simulink model "My_gfm_battery_sil_2"  (R2018b)
settings: Solver=ode45  StartTime=0.0  StopTime=30  MaxStep=1e-4  RelTol=1e-3
PreLoadFcn:
  | modelDir = fileparts(get_param(bdroot,'FileName'));
  | 
  | load_system(fullfile(modelDir,'controls_element_lib.slx'));
  | load_system(fullfile(modelDir,'test_sequence_lib.slx'));
InitFcn:
  | close all;
  | clear all;
  | clc;
  | 
  | % frequency nominals
  | F_NOM = 60;
  | W_NOM = 2 * pi * F_NOM;
  | 
  | % base values relative to inverter
  | % --------------------------------
  | VLL_INV_NOM = 480;
  | P_INV_NOM = 1e6;
  | Q_INV_NOM = 0.5e6;
  | S_INV_NOM = sqrt(P_INV_NOM^2 + Q_INV_NOM^2);
  | 
  | I_INV_BASE = S_INV_NOM/(sqrt(3)*VLL_INV_NOM);
  | Z_INV_BASE = VLL_INV_NOM^2/S_INV_NOM;
  | L_INV_BASE = Z_INV_BASE / W_NOM;
  | C_INV_BASE = 1 / (Z_INV_BASE * W_NOM);
  | 
  | % nominal ratings for Plant model
  | % --------------------------------------
  | INVERTER_COUNT = 100;
  | 
  | VLV_NOM = VLL_INV_NOM;
  | VMV_NOM = 35e3;
  | VHV_NOM = 230e3;
  | S_PLANT = INVERTER_COUNT * S_INV_NOM;
  | 
  | N_GSU = VHV_NOM/VMV_NOM;
  | N_MVT = VMV_NOM/VLV_NOM;
  | 
  | I_LV_BASE = S_PLANT/(sqrt(3)*VLV_NOM);
  | I_MV_BASE = S_PLANT/(sqrt(3)*VMV_NOM);
  | I_HV_BASE = S_PLANT/(sqrt(3)*VHV_NOM);
  | 
  | Z_LV_BASE = VLV_NOM^2/S_PLANT;
  | Z_MV_BASE = VMV_NOM^2/S_PLANT;
  | Z_HV_BASE = VHV_NOM^2/S_PLANT;
  | 
  | L_LV_BASE = Z_LV_BASE / W_NOM;
  | L_MV_BASE = Z_MV_BASE / W_NOM;
  | L_HV_BASE = Z_HV_BASE / W_NOM;
  | C_LV_BASE = 1 / (Z_LV_BASE * W_NOM);
  | C_MV_BASE = 1 / (Z_MV_BASE * W_NOM);
  | C_HV_BASE = 1 / (Z_HV_BASE * W_NOM);
  | 
  | % nominal ratings for Grid model
  | % --------------------------------------
  | VGRID_NOM = VHV_NOM;
  | S_GRID = 2*S_PLANT;
  | I_HV_BASE = S_GRID/(sqrt(3)*VGRID_NOM);
  | Z_GRID_BASE = VGRID_NOM^2/S_GRID;
  | L_GRID_BASE = Z_GRID_BASE / W_NOM;
  | C_GRID_BASE = 1 / (Z_GRID_BASE * W_NOM);
undefined symbols (not defined in the file): j
libraries: simulink x74, controls_element_lib x20, test_sequence_lib x12
(part 5 of 9)

== system My_gfm_battery_sil_2/My Inverter Controller /My_acChecks_A_V3/Clear Timer5 ==
  note: Max one sample delay on Rise
  note: Min one sample delay on Fall
  in : Inport
  Constant : Constant  Value=T_STEP
  Constant1 : Constant  Value=0
  Constant2 : Constant  Value=TIMEOUT
  Constant3 : Constant  Value=T_STEP
  Min1 : MinMax  Function=max  Inputs=2
  Min2 : MinMax  Function=max  Inputs=2
  Relational Operator : RelationalOperator  Operator=>  OutDataTypeStr=boolean  RndMeth=Simplest
  Sum1 : Sum  Inputs=|++
  Sum2 : Sum  Inputs=|-+
  Switch : Switch  Criteria=u2 > Threshold
  Unit Delay : UnitDelay  InitialCondition=TIMER_INIT  SampleTime=T_STEP
  out : Outport  VectorParamsAs1DForOutWhenUnconnected=on
  wires:
  Sum1/1 -> Switch/1
  Sum2/1 -> Relational Operator/1, Min2/1
  Constant/1 -> Sum2/1
  Min2/1 -> Switch/3
  Constant1/1 -> Min2/2, Relational Operator/2
  Unit Delay/1 -> Sum2/2
  in/1 -> Switch/2
  Switch/1 -> Unit Delay/1
  Relational Operator/1 -> out/1
  Constant2/1 -> Min1/1
  Constant3/1 -> Min1/2, Sum1/2
  Min1/1 -> Sum1/1

== system My_gfm_battery_sil_2/My Inverter Controller /My_acChecks_A_V3/Clear Timer6 ==
  note: Max one sample delay on Rise
  note: Min one sample delay on Fall
  in : Inport
  Constant : Constant  Value=T_STEP
  Constant1 : Constant  Value=0
  Constant2 : Constant  Value=TIMEOUT
  Constant3 : Constant  Value=T_STEP
  Min1 : MinMax  Function=max  Inputs=2
  Min2 : MinMax  Function=max  Inputs=2
  Relational Operator : RelationalOperator  Operator=>  OutDataTypeStr=boolean  RndMeth=Simplest
  Sum1 : Sum  Inputs=|++
  Sum2 : Sum  Inputs=|-+
  Switch : Switch  Criteria=u2 > Threshold
  Unit Delay : UnitDelay  InitialCondition=TIMER_INIT  SampleTime=T_STEP
  out : Outport  VectorParamsAs1DForOutWhenUnconnected=on
  wires:
  Sum1/1 -> Switch/1
  Sum2/1 -> Relational Operator/1, Min2/1
  Constant/1 -> Sum2/1
  Min2/1 -> Switch/3
  Constant1/1 -> Min2/2, Relational Operator/2
  Unit Delay/1 -> Sum2/2
  in/1 -> Switch/2
  Switch/1 -> Unit Delay/1
  Relational Operator/1 -> out/1
  Constant2/1 -> Min1/1
  Constant3/1 -> Min1/2, Sum1/2
  Min1/1 -> Sum1/1

== system My_gfm_battery_sil_2/My Inverter Controller /My_acChecks_A_V3/Clear Timer7 ==
  note: Max one sample delay on Rise
  note: Min one sample delay on Fall
  in : Inport
  Constant : Constant  Value=T_STEP
  Constant1 : Constant  Value=0
  Constant2 : Constant  Value=TIMEOUT
  Constant3 : Constant  Value=T_STEP
  Min1 : MinMax  Function=max  Inputs=2
  Min2 : MinMax  Function=max  Inputs=2
  Relational Operator : RelationalOperator  Operator=>  OutDataTypeStr=boolean  RndMeth=Simplest
  Sum1 : Sum  Inputs=|++
  Sum2 : Sum  Inputs=|-+
  Switch : Switch  Criteria=u2 > Threshold
  Unit Delay : UnitDelay  InitialCondition=TIMER_INIT  SampleTime=T_STEP
  out : Outport  VectorParamsAs1DForOutWhenUnconnected=on
  wires:
  Sum1/1 -> Switch/1
  Sum2/1 -> Relational Operator/1, Min2/1
  Constant/1 -> Sum2/1
  Min2/1 -> Switch/3
  Constant1/1 -> Min2/2, Relational Operator/2
  Unit Delay/1 -> Sum2/2
  in/1 -> Switch/2
  Switch/1 -> Unit Delay/1
  Relational Operator/1 -> out/1
  Constant2/1 -> Min1/1
  Constant3/1 -> Min1/2, Sum1/2
  Min1/1 -> Sum1/1

== system My_gfm_battery_sil_2/My Inverter Controller /My_acChecks_A_V3/Clear Timer8 ==
  note: Max one sample delay on Rise
  note: Min one sample delay on Fall
  in : Inport
  Constant : Constant  Value=T_STEP
  Constant1 : Constant  Value=0
  Constant2 : Constant  Value=TIMEOUT
  Constant3 : Constant  Value=T_STEP
  Min1 : MinMax  Function=max  Inputs=2
  Min2 : MinMax  Function=max  Inputs=2
  Relational Operator : RelationalOperator  Operator=>  OutDataTypeStr=boolean  RndMeth=Simplest
  Sum1 : Sum  Inputs=|++
  Sum2 : Sum  Inputs=|-+
  Switch : Switch  Criteria=u2 > Threshold
  Unit Delay : UnitDelay  InitialCondition=TIMER_INIT  SampleTime=T_STEP
  out : Outport  VectorParamsAs1DForOutWhenUnconnected=on
  wires:
  Sum1/1 -> Switch/1
  Sum2/1 -> Relational Operator/1, Min2/1
  Constant/1 -> Sum2/1
  Min2/1 -> Switch/3
  Constant1/1 -> Min2/2, Relational Operator/2
  Unit Delay/1 -> Sum2/2
  in/1 -> Switch/2
  Switch/1 -> Unit Delay/1
  Relational Operator/1 -> out/1
  Constant2/1 -> Min1/1
  Constant3/1 -> Min1/2, Sum1/2
  Min1/1 -> Sum1/1

== system My_gfm_battery_sil_2/My Inverter Controller /My_acChecks_A_V3/Clear Timer9 ==
  note: Max one sample delay on Rise
  note: Min one sample delay on Fall
  in : Inport
  Constant : Constant  Value=T_STEP
  Constant1 : Constant  Value=0
  Constant2 : Constant  Value=TIMEOUT
  Constant3 : Constant  Value=T_STEP
  Min1 : MinMax  Function=max  Inputs=2
  Min2 : MinMax  Function=max  Inputs=2
  Relational Operator : RelationalOperator  Operator=>  OutDataTypeStr=boolean  RndMeth=Simplest
  Sum1 : Sum  Inputs=|++
  Sum2 : Sum  Inputs=|-+
  Switch : Switch  Criteria=u2 > Threshold
  Unit Delay : UnitDelay  InitialCondition=TIMER_INIT  SampleTime=T_STEP
  out : Outport  VectorParamsAs1DForOutWhenUnconnected=on
  wires:
  Sum1/1 -> Switch/1
  Sum2/1 -> Relational Operator/1, Min2/1
  Constant/1 -> Sum2/1
  Min2/1 -> Switch/3
  Constant1/1 -> Min2/2, Relational Operator/2
  Unit Delay/1 -> Sum2/2
  in/1 -> Switch/2
  Switch/1 -> Unit Delay/1
  Relational Operator/1 -> out/1
  Constant2/1 -> Min1/1
  Constant3/1 -> Min1/2, Sum1/2
  Min1/1 -> Sum1/1

== system My_gfm_battery_sil_2/My Inverter Controller /My_acChecks_A_V3/OF1 Timer ==
  note: Min one sample delay on Rise
  note: Max one sample delay on Fall
  in : Inport
  Constant : Constant  Value=T_STEP
  Constant1 : Constant  Value=0
  Constant2 : Constant  Value=TIMEOUT
  Constant3 : Constant  Value=T_STEP
  Gain : Gain  Gain=0
  Min1 : MinMax  Function=max  Inputs=2
  Min2 : MinMax  Inputs=2
  Relational Operator : RelationalOperator  Operator=>  OutDataTypeStr=boolean  RndMeth=Simplest
  Sum1 : Sum  Inputs=|++
  Sum2 : Sum  Inputs=|++
  Switch : Switch  Criteria=u2 > Threshold
  Unit Delay : UnitDelay  SampleTime=T_STEP
  out : Outport  VectorParamsAs1DForOutWhenUnconnected=on
  wires:
  Sum2/1 -> Relational Operator/1, Min2/1
  Sum1/1 -> Min2/2, Relational Operator/2
  Constant/1 -> Sum2/1
  Min2/1 -> Switch/1
  Constant1/1 -> Switch/3
  Unit Delay/1 -> Sum2/2
  in/1 -> Switch/2
  Switch/1 -> Unit Delay/1
  Relational Operator/1 -> out/1
  Min1/1 -> Sum1/1
  Constant2/1 -> Min1/1
  Constant3/1 -> Min1/2, Gain/1
  Gain/1 -> Sum1/2

== system My_gfm_battery_sil_2/My Inverter Controller /My_acChecks_A_V3/OF2 Timer ==
  note: Min one sample delay on Rise
  note: Max one sample delay on Fall
  in : Inport
  Constant : Constant  Value=T_STEP
  Constant1 : Constant  Value=0
  Constant2 : Constant  Value=TIMEOUT
  Constant3 : Constant  Value=T_STEP
  Gain : Gain  Gain=0
  Min1 : MinMax  Function=max  Inputs=2
  Min2 : MinMax  Inputs=2
  Relational Operator : RelationalOperator  Operator=>  OutDataTypeStr=boolean  RndMeth=Simplest
  Sum1 : Sum  Inputs=|++
  Sum2 : Sum  Inputs=|++
  Switch : Switch  Criteria=u2 > Threshold
  Unit Delay : UnitDelay  SampleTime=T_STEP
  out : Outport  VectorParamsAs1DForOutWhenUnconnected=on
  wires:
  Sum2/1 -> Relational Operator/1, Min2/1
  Sum1/1 -> Min2/2, Relational Operator/2
  Constant/1 -> Sum2/1
  Min2/1 -> Switch/1
  Constant1/1 -> Switch/3
  Unit Delay/1 -> Sum2/2
  in/1 -> Switch/2
  Switch/1 -> Unit Delay/1
  Relational Operator/1 -> out/1
  Min1/1 -> Sum1/1
  Constant2/1 -> Min1/1
  Constant3/1 -> Min1/2, Gain/1
  Gain/1 -> Sum1/2

== system My_gfm_battery_sil_2/My Inverter Controller /My_acChecks_A_V3/OF3 Timer ==
  note: Min one sample delay on Rise
  note: Max one sample delay on Fall
  in : Inport
  Constant : Constant  Value=T_STEP
  Constant1 : Constant  Value=0
  Constant2 : Constant  Value=TIMEOUT
  Constant3 : Constant  Value=T_STEP
  Gain : Gain  Gain=0
  Min1 : MinMax  Function=max  Inputs=2
  Min2 : MinMax  Inputs=2
  Relational Operator : RelationalOperator  Operator=>  OutDataTypeStr=boolean  RndMeth=Simplest
  Sum1 : Sum  Inputs=|++
  Sum2 : Sum  Inputs=|++
  Switch : Switch  Criteria=u2 > Threshold
  Unit Delay : UnitDelay  SampleTime=T_STEP
  out : Outport  VectorParamsAs1DForOutWhenUnconnected=on
  wires:
  Sum2/1 -> Relational Operator/1, Min2/1
  Sum1/1 -> Min2/2, Relational Operator/2
  Constant/1 -> Sum2/1
  Min2/1 -> Switch/1
  Constant1/1 -> Switch/3
  Unit Delay/1 -> Sum2/2
  in/1 -> Switch/2
  Switch/1 -> Unit Delay/1
  Relational Operator/1 -> out/1
  Min1/1 -> Sum1/1
  Constant2/1 -> Min1/1
  Constant3/1 -> Min1/2, Gain/1
  Gain/1 -> Sum1/2

== system My_gfm_battery_sil_2/My Inverter Controller /My_acChecks_A_V3/OV1 Timer ==
  note: Min one sample delay on Rise
  note: Max one sample delay on Fall
  in : Inport
  Constant : Constant  Value=T_STEP
  Constant1 : Constant  Value=0
  Constant2 : Constant  Value=TIMEOUT
  Constant3 : Constant  Value=T_STEP
  Gain : Gain  Gain=0
  Min1 : MinMax  Function=max  Inputs=2
  Min2 : MinMax  Inputs=2
  Relational Operator : RelationalOperator  Operator=>  OutDataTypeStr=boolean  RndMeth=Simplest
  Sum1 : Sum  Inputs=|++
  Sum2 : Sum  Inputs=|++
  Switch : Switch  Criteria=u2 > Threshold
  Unit Delay : UnitDelay  SampleTime=T_STEP
  out : Outport  VectorParamsAs1DForOutWhenUnconnected=on
  wires:
  Sum2/1 -> Relational Operator/1, Min2/1
  Sum1/1 -> Min2/2, Relational Operator/2
  Constant/1 -> Sum2/1
  Min2/1 -> Switch/1
  Constant1/1 -> Switch/3
  Unit Delay/1 -> Sum2/2
  in/1 -> Switch/2
  Switch/1 -> Unit Delay/1
  Relational Operator/1 -> out/1
  Min1/1 -> Sum1/1
  Constant2/1 -> Min1/1
  Constant3/1 -> Min1/2, Gain/1
  Gain/1 -> Sum1/2

== system My_gfm_battery_sil_2/My Inverter Controller /My_acChecks_A_V3/OV2 Timer ==
  note: Min one sample delay on Rise
  note: Max one sample delay on Fall
  in : Inport
  Constant : Constant  Value=T_STEP
  Constant1 : Constant  Value=0
  Constant2 : Constant  Value=TIMEOUT
  Constant3 : Constant  Value=T_STEP
  Gain : Gain  Gain=0
  Min1 : MinMax  Function=max  Inputs=2
  Min2 : MinMax  Inputs=2
  Relational Operator : RelationalOperator  Operator=>  OutDataTypeStr=boolean  RndMeth=Simplest
  Sum1 : Sum  Inputs=|++
  Sum2 : Sum  Inputs=|++
  Switch : Switch  Criteria=u2 > Threshold
  Unit Delay : UnitDelay  SampleTime=T_STEP
  out : Outport  VectorParamsAs1DForOutWhenUnconnected=on
  wires:
  Sum2/1 -> Relational Operator/1, Min2/1
  Sum1/1 -> Min2/2, Relational Operator/2
  Constant/1 -> Sum2/1
  Min2/1 -> Switch/1
  Constant1/1 -> Switch/3
  Unit Delay/1 -> Sum2/2
  in/1 -> Switch/2
  Switch/1 -> Unit Delay/1
  Relational Operator/1 -> out/1
  Min1/1 -> Sum1/1
  Constant2/1 -> Min1/1
  Constant3/1 -> Min1/2, Gain/1
  Gain/1 -> Sum1/2

== system My_gfm_battery_sil_2/My Inverter Controller /My_acChecks_A_V3/OV3 Timer ==
  note: Min one sample delay on Rise
  note: Max one sample delay on Fall
  in : Inport
  Constant : Constant  Value=T_STEP
  Constant1 : Constant  Value=0
  Constant2 : Constant  Value=TIMEOUT
  Constant3 : Constant  Value=T_STEP
  Gain : Gain  Gain=0
  Min1 : MinMax  Function=max  Inputs=2
  Min2 : MinMax  Inputs=2
  Relational Operator : RelationalOperator  Operator=>  OutDataTypeStr=boolean  RndMeth=Simplest
  Sum1 : Sum  Inputs=|++
  Sum2 : Sum  Inputs=|++
  Switch : Switch  Criteria=u2 > Threshold
  Unit Delay : UnitDelay  SampleTime=T_STEP
  out : Outport  VectorParamsAs1DForOutWhenUnconnected=on
  wires:
  Sum2/1 -> Relational Operator/1, Min2/1
  Sum1/1 -> Min2/2, Relational Operator/2
  Constant/1 -> Sum2/1
  Min2/1 -> Switch/1
  Constant1/1 -> Switch/3
  Unit Delay/1 -> Sum2/2
  in/1 -> Switch/2
  Switch/1 -> Unit Delay/1
  Relational Operator/1 -> out/1
  Min1/1 -> Sum1/1
  Constant2/1 -> Min1/1
  Constant3/1 -> Min1/2, Gain/1
  Gain/1 -> Sum1/2

== system My_gfm_battery_sil_2/My Inverter Controller /My_acChecks_A_V3/UF1 Timer ==
  note: Min one sample delay on Rise
  note: Max one sample delay on Fall
  in : Inport
  Constant : Constant  Value=T_STEP
  Constant1 : Constant  Value=0
  Constant2 : Constant  Value=TIMEOUT
  Constant3 : Constant  Value=T_STEP
  Gain : Gain  Gain=0
  Min1 : MinMax  Function=max  Inputs=2
  Min2 : MinMax  Inputs=2
  Relational Operator : RelationalOperator  Operator=>  OutDataTypeStr=boolean  RndMeth=Simplest
  Sum1 : Sum  Inputs=|++
  Sum2 : Sum  Inputs=|++
  Switch : Switch  Criteria=u2 > Threshold
  Unit Delay : UnitDelay  SampleTime=T_STEP
  out : Outport  VectorParamsAs1DForOutWhenUnconnected=on
  wires:
  Sum2/1 -> Relational Operator/1, Min2/1
  Sum1/1 -> Min2/2, Relational Operator/2
  Constant/1 -> Sum2/1
  Min2/1 -> Switch/1
  Constant1/1 -> Switch/3
  Unit Delay/1 -> Sum2/2
  in/1 -> Switch/2
  Switch/1 -> Unit Delay/1
  Relational Operator/1 -> out/1
  Min1/1 -> Sum1/1
  Constant2/1 -> Min1/1
  Constant3/1 -> Min1/2, Gain/1
  Gain/1 -> Sum1/2

== system My_gfm_battery_sil_2/My Inverter Controller /My_acChecks_A_V3/UF2 Timer ==
  note: Min one sample delay on Rise
  note: Max one sample delay on Fall
  in : Inport
  Constant : Constant  Value=T_STEP
  Constant1 : Constant  Value=0
  Constant2 : Constant  Value=TIMEOUT
  Constant3 : Constant  Value=T_STEP
  Gain : Gain  Gain=0
  Min1 : MinMax  Function=max  Inputs=2
  Min2 : MinMax  Inputs=2
  Relational Operator : RelationalOperator  Operator=>  OutDataTypeStr=boolean  RndMeth=Simplest
  Sum1 : Sum  Inputs=|++
  Sum2 : Sum  Inputs=|++
  Switch : Switch  Criteria=u2 > Threshold
  Unit Delay : UnitDelay  SampleTime=T_STEP
  out : Outport  VectorParamsAs1DForOutWhenUnconnected=on
  wires:
  Sum2/1 -> Relational Operator/1, Min2/1
  Sum1/1 -> Min2/2, Relational Operator/2
  Constant/1 -> Sum2/1
  Min2/1 -> Switch/1
  Constant1/1 -> Switch/3
  Unit Delay/1 -> Sum2/2
  in/1 -> Switch/2
  Switch/1 -> Unit Delay/1
  Relational Operator/1 -> out/1
  Min1/1 -> Sum1/1
  Constant2/1 -> Min1/1
  Constant3/1 -> Min1/2, Gain/1
  Gain/1 -> Sum1/2

== system My_gfm_battery_sil_2/My Inverter Controller /My_acChecks_A_V3/UF3 Timer ==
  note: Min one sample delay on Rise
  note: Max one sample delay on Fall
  in : Inport
  Constant : Constant  Value=T_STEP
  Constant1 : Constant  Value=0
  Constant2 : Constant  Value=TIMEOUT
  Constant3 : Constant  Value=T_STEP
  Gain : Gain  Gain=0
  Min1 : MinMax  Function=max  Inputs=2
  Min2 : MinMax  Inputs=2
  Relational Operator : RelationalOperator  Operator=>  OutDataTypeStr=boolean  RndMeth=Simplest
  Sum1 : Sum  Inputs=|++
  Sum2 : Sum  Inputs=|++
  Switch : Switch  Criteria=u2 > Threshold
  Unit Delay : UnitDelay  SampleTime=T_STEP
  out : Outport  VectorParamsAs1DForOutWhenUnconnected=on
  wires:
  Sum2/1 -> Relational Operator/1, Min2/1
  Sum1/1 -> Min2/2, Relational Operator/2
  Constant/1 -> Sum2/1
  Min2/1 -> Switch/1
  Constant1/1 -> Switch/3
  Unit Delay/1 -> Sum2/2
  in/1 -> Switch/2
  Switch/1 -> Unit Delay/1
  Relational Operator/1 -> out/1
  Min1/1 -> Sum1/1
  Constant2/1 -> Min1/1
  Constant3/1 -> Min1/2, Gain/1
  Gain/1 -> Sum1/2

== system My_gfm_battery_sil_2/My Inverter Controller /My_acChecks_A_V3/UV1 Timer ==
  note: Min one sample delay on Rise
  note: Max one sample delay on Fall
  in : Inport
  Constant : Constant  Value=T_STEP
  Constant1 : Constant  Value=0
  Constant2 : Constant  Value=TIMEOUT
  Constant3 : Constant  Value=T_STEP
  Gain : Gain  Gain=0
  Min1 : MinMax  Function=max  Inputs=2
  Min2 : MinMax  Inputs=2
  Relational Operator : RelationalOperator  Operator=>  OutDataTypeStr=boolean  RndMeth=Simplest
  Sum1 : Sum  Inputs=|++
  Sum2 : Sum  Inputs=|++
  Switch : Switch  Criteria=u2 > Threshold
  Unit Delay : UnitDelay  SampleTime=T_STEP
  out : Outport  VectorParamsAs1DForOutWhenUnconnected=on
  wires:
  Sum2/1 -> Relational Operator/1, Min2/1
  Sum1/1 -> Min2/2, Relational Operator/2
  Constant/1 -> Sum2/1
  Min2/1 -> Switch/1
  Constant1/1 -> Switch/3
  Unit Delay/1 -> Sum2/2
  in/1 -> Switch/2
  Switch/1 -> Unit Delay/1
  Relational Operator/1 -> out/1
  Min1/1 -> Sum1/1
  Constant2/1 -> Min1/1
  Constant3/1 -> Min1/2, Gain/1
  Gain/1 -> Sum1/2

== system My_gfm_battery_sil_2/My Inverter Controller /My_acChecks_A_V3/UV2 Timer ==
  note: Min one sample delay on Rise
  note: Max one sample delay on Fall
  in : Inport
  Constant : Constant  Value=T_STEP
  Constant1 : Constant  Value=0
  Constant2 : Constant  Value=TIMEOUT
  Constant3 : Constant  Value=T_STEP
  Gain : Gain  Gain=0
  Min1 : MinMax  Function=max  Inputs=2
  Min2 : MinMax  Inputs=2
  Relational Operator : RelationalOperator  Operator=>  OutDataTypeStr=boolean  RndMeth=Simplest
  Sum1 : Sum  Inputs=|++
  Sum2 : Sum  Inputs=|++
  Switch : Switch  Criteria=u2 > Threshold
  Unit Delay : UnitDelay  SampleTime=T_STEP
  out : Outport  VectorParamsAs1DForOutWhenUnconnected=on
  wires:
  Sum2/1 -> Relational Operator/1, Min2/1
  Sum1/1 -> Min2/2, Relational Operator/2
  Constant/1 -> Sum2/1
  Min2/1 -> Switch/1
  Constant1/1 -> Switch/3
  Unit Delay/1 -> Sum2/2
  in/1 -> Switch/2
  Switch/1 -> Unit Delay/1
  Relational Operator/1 -> out/1
  Min1/1 -> Sum1/1
  Constant2/1 -> Min1/1
  Constant3/1 -> Min1/2, Gain/1
  Gain/1 -> Sum1/2

== system My_gfm_battery_sil_2/My Inverter Controller /My_acChecks_A_V3/UV3 Timer ==
  note: Min one sample delay on Rise
  note: Max one sample delay on Fall
  in : Inport
  Constant : Constant  Value=T_STEP
  Constant1 : Constant  Value=0
  Constant2 : Constant  Value=TIMEOUT
  Constant3 : Constant  Value=T_STEP
  Gain : Gain  Gain=0
  Min1 : MinMax  Function=max  Inputs=2
  Min2 : MinMax  Inputs=2
  Relational Operator : RelationalOperator  Operator=>  OutDataTypeStr=boolean  RndMeth=Simplest
  Sum1 : Sum  Inputs=|++
  Sum2 : Sum  Inputs=|++
  Switch : Switch  Criteria=u2 > Threshold
  Unit Delay : UnitDelay  SampleTime=T_STEP
  out : Outport  VectorParamsAs1DForOutWhenUnconnected=on
  wires:
  Sum2/1 -> Relational Operator/1, Min2/1
  Sum1/1 -> Min2/2, Relational Operator/2
  Constant/1 -> Sum2/1
  Min2/1 -> Switch/1
  Constant1/1 -> Switch/3
  Unit Delay/1 -> Sum2/2
  in/1 -> Switch/2
  Switch/1 -> Unit Delay/1
  Relational Operator/1 -> out/1
  Min1/1 -> Sum1/1
  Constant2/1 -> Min1/1
  Constant3/1 -> Min1/2, Gain/1
  Gain/1 -> Sum1/2

== system My_gfm_battery_sil_2/My Inverter Controller /My_acMonitor_A/Analyzer_V ==
  note: What is that?
  note: complex multiplication
  note: Let
      | V+*cos wt + V-*cos wt + vo * cos wt + vdc
      | V+*cos (wt-120) + V-*cos (wt+120) vo * cos wt + vdc
      | V+*cos (wt+120) + V-*cos (wt-120) vo * cos wt + vdc
  note: filter to remove pulsating on whatever
      | a frame coming from opposie rotating
  note: + conj
  note: Vd- , Vq-
  note: Vd+ , Vq+
  note: - conj
  note: Not sure why SOGI filter was not used
      | to get clean Pve and Nve
  note: cos x + j sin x
      | cos (x-120) + j (sin x -120)
      | cos (x+120) + j (sin x +120)
  note: cos x - j sin x
  note: V+/2*[1+cos2wt] + V-/2*[1+cos2wt] + vo/2*[1+cos2wt] + vdc * cos wt
      | V+/2*[cos(2pi/3)+cos(2wt-2pi/3)] + V-/2*[cos(2pi/3)+cos(2wt-4pi/3)] + vo/2*[1+cos2wt] + vdc * cos wt
      | V+/2*[cos(2pi/3)+cos(2wt-4pi/3)] + V-/2*[cos(2pi/3)+cos(2wt-2pi/3)] + vo/2*[1+cos2wt] + vdc * cos wt
      |
      | -V+/2*[sin2wt] - V-/2*[sin2wt] - vo/2*[sin2wt] - vdc * sin wt
      | -V+/2*[sin(2wt-2pi/3)+sin(2pi/3)] - V-/2*[sin(2wt-4pi/3)-sin(2pi/3)] - vo/2*[sin2wt] - vdc * sin wt
      | -V+/2*[sin(2wt-4pi/3)-sin(2pi/3)] - V-/2*[sin(2wt-2pi/3)+sin(2pi/3)] - vo/2*[sin2wt] - vdc * sin wt
  note: [ 1 ]
      | [ exp(- j2pi/3)]
      | [ exp(- j4pi/3)]
  note: [ 1 ]
      | [ exp(- j4pi/3)]
      | [ exp(- j8pi/3)] = [ exp(- j2pi/3)]
  note: Remove double frequency
      | V+/2+ V-/2+ vo/2 + vdc*coswt
      | V+/2*cos(2pi/3) + V-/2*cos(2pi/3) + vo/2 + vdc*coswt
      | V+/2*cos(2pi/3) + V-/2*cos(2pi/3) + vo/2 + vdc*coswt
      |
      | - vdc*sinwt
      | -V+/2*sin(2pi/3) - V-/2*-sin(2pi/3) - vdc*sinwt
      | -V+/2*-sin(2pi/3) - V-/2*+sin(2pi/3) - vdc*sinwt
  note: sqrt(2) *[V+/2+ V-/2+ vo/2 + vdc*coswt]
      | sqrt(2) *[V+/2*cos(2pi/3) + V-/2*cos(2pi/3) + vo/2 + vdc*coswt]
      | sqrt(2) *[V+/2*cos(2pi/3) + V-/2*cos(2pi/3) + vo/2 + vdc*coswt]
      |
      | sqrt(2) *[- vdc*sinwt]
      | sqrt(2) *[-V+/2*sin(2pi/3) - V-/2*-sin(2pi/3) - vdc*sinwt]
      | sqrt(2) *[-V+/2*-sin(2pi/3) - V-/2*+sin(2pi/3) - vdc*sinwt]
  note: 1
      | cos(-4pi/3)
      | cos(-2pi/3)
      |
      | 0
      | sin(-4pi/3)
      | sin(-2pi/3)
  note: 1
      | cos(-2pi/3)
      | cos(-4pi/3)
      |
      | 0
      | sin(-2pi/3)
      | sin(-4pi/3)
  note: sqrt(2) *[V+/2+ V-/2+ vo/2 + vdc*coswt] * 1 - sqrt(2) *[- vdc*sinwt] * 0
      | sqrt(2) *[V+/2*cos(2pi/3) + V-/2*cos(2pi/3) + vo/2 + vdc*coswt] * cos(-4pi/3) - sqrt(2) *[-V+/2*sin(2pi/3) - V-/2*-sin(2pi/3) - vdc*sinwt] * sin(-4pi/3)
      | sqrt(2) *[V+/2*cos(2pi/3) + V-/2*cos(2pi/3) + vo/2 + vdc*coswt] * cos(-2pi/3) - sqrt(2) *[-V+/2*-sin(2pi/3) - V-/2*+sin(2pi/3) - vdc*sinwt] * sin(-2pi/3)
      |
      | sqrt(2) *[V+/2+ V-/2+ vo/2 + vdc*coswt] * 0 + sqrt(2) *[- vdc*sinwt] * 1
      | sqrt(2) *[V+/2*cos(2pi/3) + V-/2*cos(2pi/3) + vo/2 + vdc*coswt] * sin(-4pi/3) + sqrt(2) *[-V+/2*sin(2pi/3) - V-/2*-sin(2pi/3) - vdc*sinwt] * cos(-4pi/3)
      | sqrt(2) *[V+/2*cos(2pi/3) + V-/2*cos(2pi/3) + vo/2 + vdc*coswt] * sin(-2pi/3) + sqrt(2) *[-V+/2*-sin(2pi/3) - V-/2*+sin(2pi/3) - vdc*sinwt] * cos(-2pi/3)
  note: 3 * sqrt(2) *[vo/2 + vdc*coswt]
      |
      | 3 * sqrt(2) *[- vdc*sinwt]
  note: sqrt(2) *[vo/2 + vdc*coswt]
      |
      | sqrt(2) *[- vdc*sinwt]
  note: sqrt(2) *[V+/2+ V-/2+ vo/2 + vdc*coswt]
      | sqrt(2) *[V+/2*-0.5 + V-/2*-0.5 + vo/2 + vdc*coswt] * -0.5 - sqrt(2) *[-V+/2*sqrt(3/2) - V-/2*-sqrt(3/2) - vdc*sinwt] * sqrt(3/2)
      | sqrt(2) *[V+/2*-0.5 + V-/2*-0.5 + vo/2 + vdc*coswt] * -0.5 - sqrt(2) *[-V+/2*-sqrt(3/2) - V-/2*+sqrt(3/2) - vdc*sinwt] * -sqrt(3/2)
      |
      | sqrt(2) *[V+/2+ V-/2+ vo/2 + vdc*coswt] * 0 + sqrt(2) *[- vdc*sinwt] * 1
      | sqrt(2) *[V+/2* -0.5 + V-/2* -0.5 + vo/2 + vdc*coswt] * sqrt(3/2) + sqrt(2) *[-V+/2* sqrt(3/2) - V-/2*- sqrt(3/2) - vdc*sinwt] * -0.5
      | sqrt(2) *[V+/2* -0.5 + V-/2* -0.5 + vo/2 + vdc*coswt] * - sqrt(3/2) + sqrt(2) *[-V+/2*- sqrt(3/2) - V-/2* sqrt(3/2) - vdc*sinwt] * -0.5
  note: sqrt(2) *[3 * V+/2+ 0 * V-/2+ 0 * vo/2 + 0 * vdc*coswt
      |
      | sqrt(2) *[0 * V+/2+ 0 * V-/2+ 0 * vo/2 + 0 * vdc*coswt
  note: sqrt(2) *[V+/2]
      |
      | 0
  note: sqrt(3) * sqrt(2) *[V+/2]
      |
      | 0
  note: sqrt(3) *sqrt(2) *[vo/2 + vdc*coswt]
      |
      | sqrt(3)* sqrt(2) *[- vdc*sinwt]
  note: sqrt(2) *[V+/2+ V-/2+ vo/2 + vdc*coswt] * 1 - sqrt(2) *[- vdc*sinwt] * 0
      | sqrt(2) *[V+/2*cos(2pi/3) + V-/2*cos(2pi/3) + vo/2 + vdc*coswt] * cos(-2pi/3) - sqrt(2) *[-V+/2*sin(2pi/3) - V-/2*-sin(2pi/3) - vdc*sinwt] * sin(-2pi/3)
      | sqrt(2) *[V+/2*cos(2pi/3) + V-/2*cos(2pi/3) + vo/2 + vdc*coswt] * cos(-4pi/3) - sqrt(2) *[-V+/2*-sin(2pi/3) - V-/2*+sin(2pi/3) - vdc*sinwt] * sin(-4pi/3)
      |
      | sqrt(2) *[V+/2+ V-/2+ vo/2 + vdc*coswt] * 0 + sqrt(2) *[- vdc*sinwt] * 1
      | sqrt(2) *[V+/2*cos(2pi/3) + V-/2*cos(2pi/3) + vo/2 + vdc*coswt] * sin(-2pi/3) + sqrt(2) *[-V+/2*sin(2pi/3) - V-/2*-sin(2pi/3) - vdc*sinwt] * cos(-2pi/3)
      | sqrt(2) *[V+/2*cos(2pi/3) + V-/2*cos(2pi/3) + vo/2 + vdc*coswt] * sin(-4pi/3) + sqrt(2) *[-V+/2*-sin(2pi/3) - V-/2*+sin(2pi/3) - vdc*sinwt] * cos(-4pi/3)
  note: sqrt(2) *[V+/2+ V-/2+ vo/2 + vdc*coswt]
      | sqrt(2) *[V+/2*-0.5 + V-/2*-0.5 + vo/2 + vdc*coswt] * -0.5 - sqrt(2) *[-V+/2*sqrt(3/2) - V-/2*-sqrt(3/2) - vdc*sinwt] * -sqrt(3/2)
      | sqrt(2) *[V+/2*-0.5 + V-/2*-0.5 + vo/2 + vdc*coswt] * -0.5 - sqrt(2) *[-V+/2*-sqrt(3/2) - V-/2*+sqrt(3/2) - vdc*sinwt] * sqrt(3/2)
      |
      | sqrt(2) *[V+/2+ V-/2+ vo/2 + vdc*coswt] * 0 + sqrt(2) *[- vdc*sinwt] * 1
      | sqrt(2) *[V+/2*-0.5 + V-/2*-0.5 + vo/2 + vdc*coswt] * -sqrt(3/2) + sqrt(2) *[-V+/2*sqrt(3/2) - V-/2*-sqrt(3/2) - vdc*sinwt] * -0.5
      | sqrt(2) *[V+/2*-0.5 + V-/2*-0.5 + vo/2 + vdc*coswt] * sqrt(3/2) + sqrt(2) *[-V+/2*-sqrt(3/2) - V-/2*sqrt(3/2) - vdc*sinwt] * -0.5
  note: sqrt(2) *[0 * V+/2+ 3 * V-/2+ 0 * vo/2 + 0 * vdc*coswt
      |
      | sqrt(2) *[0 * V+/2+ 0 * V-/2+ 0 * vo/2 + 0 * vdc*coswt
  note: sqrt(2) *[V-/2]
      |
      | 0
  note: sqrt(3) *sqrt(2) *[V-/2]
      |
      | 0
  note: sqrt(2) *[V+/2+ V-/2+ vo/2 + vdc*coswt]
      | sqrt(2) *[V+/2*cos(2pi/3) + V-/2*cos(2pi/3) + vo/2 + vdc*coswt] * cos(-4pi/3) - sqrt(2) *[-V+/2*sin(2pi/3) - V-/2*-sin(2pi/3) - vdc*sinwt] * sin(-4pi/3)
      | sqrt(2) *[V+/2*cos(2pi/3) + V-/2*cos(2pi/3) + vo/2 + vdc*coswt] * cos(-2pi/3) - sqrt(2) *[-V+/2*-sin(2pi/3) - V-/2*+sin(2pi/3) - vdc*sinwt] * sin(-2pi/3)
      |
      | sqrt(2) *[- vdc*sinwt]
      | sqrt(2) *[V+/2*cos(2pi/3) + V-/2*cos(2pi/3) + vo/2 + vdc*coswt] * sin(-4pi/3) + sqrt(2) *[-V+/2*sin(2pi/3) - V-/2*-sin(2pi/3) - vdc*sinwt] * cos(-4pi/3)
      | sqrt(2) *[V+/2*cos(2pi/3) + V-/2*cos(2pi/3) + vo/2 + vdc*coswt] * sin(-2pi/3) + sqrt(2) *[-V+/2*-sin(2pi/3) - V-/2*+sin(2pi/3) - vdc*sinwt] * cos(-2pi/3)
  in[3] : Inport
  osc[3] : Inport  Port=2
  Conj : Math  Operator=conj  SaturateOnIntegerOverflow=on
  Demux : Demux  Outputs=3
  Gain2 : Gain  Gain=1/3
  Gain3 : Gain  Gain=1/3
  Gain4 : Gain  Gain=1/3
  Gain5 : Gain  Gain=sqrt(2)
  Product1 : Product
  Product2 : Product
  Product3 : Product
  Rotation : Constant  Value=exp(j*2*pi*[0 -1/3 -2/3])
  Rotation1 : Constant  Value=exp(j*2*pi*[0 -1/3 -2/3])
  Square : Math  Operator=square  SaturateOnIntegerOverflow=on
  Sum of Elements1 : Sum  Inputs=+
  Sum of Elements2 : Sum  Inputs=+
  Sum of Elements3 : Sum  Inputs=+
  Terminator : Terminator
  Terminator1 : Terminator
  complex_LPF : Subsystem  mask{tau=0.05}
      mask prompts: tau "Time constant"
  convert_to_LL : Gain  Gain=sqrt(3)
  convert_to_LL1 : Gain  Gain=sqrt(3)
  convert_to_LL2 : Gain  Gain=sqrt(3)
  fund[3] : Outport  VectorParamsAs1DForOutWhenUnconnected=on
  Zero : Outport  Port=2  VectorParamsAs1DForOutWhenUnconnected=on
  Pve : Outport  Port=3  VectorParamsAs1DForOutWhenUnconnected=on
  Nve : Outport  Port=4  VectorParamsAs1DForOutWhenUnconnected=on
  wires:
  convert_to_LL2/1 -> Nve/1
  convert_to_LL1/1 -> Pve/1
  convert_to_LL/1 -> Zero/1
  Gain4/1 -> convert_to_LL2/1
  complex_LPF/1(Out1) -> Gain5/1
  Product3/1 -> Sum of Elements3/1
  Product1/1 -> complex_LPF/1(In1)
  Demux/1 -> Conj/1
  Rotation/1 -> Square/1
  Rotation1/1 -> Product3/2
  Sum of Elements2/1 -> Gain3/1
  Conj/1 -> Product1/2
  Sum of Elements1/1 -> Gain2/1
  Square/1 -> Product2/2
  Sum of Elements3/1 -> Gain4/1
  osc[3]/1 -> Demux/1
  Gain3/1 -> convert_to_LL1/1
  Gain2/1 -> convert_to_LL/1
  in[3]/1 -> Product1/1
  Demux/2 -> Terminator/1
  Demux/3 -> Terminator1/1
  Gain5/1 -> Sum of Elements1/1, Product3/1, Product2/1
  Product2/1 -> Sum of Elements2/1, fund[3]/1

== system My_gfm_battery_sil_2/My Inverter Controller /My_acMonitor_A/Analyzer_V1 ==
  note: Let Va coswt, so
      | V/2 *[ exp(jw) +exp(-jw)]
      | V/2 *[ exp(jw - j2pi/3) +exp(-jw + j2pi/3)]
      | V/2 *[ exp(jw - j4pi/3) +exp(-jw + j4pi/3)]
  note: filter to remove pulsating on whatever
      | a frame coming from opposie rotating
  note: + conj
  note: Vd- , Vq-
  note: Vd+ , Vq+
  note: - conj
  note: Not sure why SOGI filter was not used
      | to get clean Pve and Nve
  note: cos x + j sin x
      | cos (x-120) + j (sin x -120)
      | cos (x+120) + j (sin x +120)
  note: cos x - j sin x
  note: V/2 *[ 1 +exp(-2jw)]
      | V/2 *[ exp(- j2pi/3) +exp(-2jw + j2pi/3)]
      | V/2 *[ exp(- j4pi/3) +exp(-2jw + j4pi/3)]
  note: Remove double frequency
      | V/2 *[ 1 ]
      | V/2 *[ exp(- j2pi/3)]
      | V/2 *[ exp(- j4pi/3)]
  note: sqrt(2) * V/2 *[ 1 ]
      | sqrt(2) * V/2 *[ exp(- j2pi/3)]
      | sqrt(2) * V/2 *[ exp(- j4pi/3)]
  note: [ 1 ]
      | [ exp(- j2pi/3)]
      | [ exp(- j4pi/3)]
  note: sqrt(2) * V/2 *[ 1 ]
      | sqrt(2) * V/2 *[ exp(- j4pi/3)]
      | sqrt(2) * V/2 *[ exp(- j8pi/3)] = sqrt(2) * V/2 *[ exp(- j2pi/3)]
  note: [ 1 ]
      | [ exp(- j4pi/3)]
      | [ exp(- j8pi/3)] = [ exp(- j2pi/3)]
  note: sqrt(2) * V/2 *[ 1 ]
      | sqrt(2) * V/2 *[ exp(- j6pi/3)] = sqrt(2) * Vb/2
      | sqrt(2) * V/2 *[ exp(- j6pi/3)] = sqrt(2) * Vc/2
  note: sqrt(2) * V/2 *[ 1 ]
      | + sqrt(2) * V/2 *[ exp(- j2pi/3)]
      | + sqrt(2) * V/2 *[ exp(- j4pi/3)]
      | = 0
  note: sqrt(2) * V/2
      | + sqrt(2) * V/2
      | + sqrt(2) * V/2
      | = 3 * sqrt(2) * V/2 * 1/3 = V/sqrt(2)
      | The LN RMS
  note: sqrt(2) * V/2
      | + sqrt(2) * V/2 *[ exp(- j4pi/3)]
      | + sqrt(2) * V/2 *[ exp(- j2pi/3)]
      | = 0
      | The LN RMS
  in[3] : Inport
  osc[3] : Inport  Port=2
  Conj : Math  Operator=conj  SaturateOnIntegerOverflow=on
  Demux : Demux  Outputs=3
  Gain2 : Gain  Gain=1/3
  Gain3 : Gain  Gain=1/3
  Gain4 : Gain  Gain=1/3
  Gain5 : Gain  Gain=sqrt(2)
  Product1 : Product
  Product2 : Product
  Product3 : Product
  Rotation : Constant  Value=exp(j*2*pi*[0 -1/3 -2/3])
  Rotation1 : Constant  Value=exp(j*2*pi*[0 -1/3 -2/3])
  Square : Math  Operator=square  SaturateOnIntegerOverflow=on
  Sum of Elements1 : Sum  Inputs=+
  Sum of Elements2 : Sum  Inputs=+
  Sum of Elements3 : Sum  Inputs=+
  Terminator : Terminator
  Terminator1 : Terminator
  complex_LPF : Subsystem  mask{tau=0.05}
      mask prompts: tau "Time constant"
  convert_to_LL : Gain  Gain=sqrt(3)
  convert_to_LL1 : Gain  Gain=sqrt(3)
  convert_to_LL2 : Gain  Gain=sqrt(3)
  fund[3] : Outport  VectorParamsAs1DForOutWhenUnconnected=on
  Zero : Outport  Port=2  VectorParamsAs1DForOutWhenUnconnected=on
  Pve : Outport  Port=3  VectorParamsAs1DForOutWhenUnconnected=on
  Nve : Outport  Port=4  VectorParamsAs1DForOutWhenUnconnected=on
  wires:
  convert_to_LL2/1 -> Nve/1
  convert_to_LL1/1 -> Pve/1
  convert_to_LL/1 -> Zero/1
  Gain4/1 -> convert_to_LL2/1
  Product2/1 -> fund[3]/1, Sum of Elements2/1
  complex_LPF/1(Out1) -> Gain5/1
  Product3/1 -> Sum of Elements3/1
  Product1/1 -> complex_LPF/1(In1)
  Demux/1 -> Conj/1
  Rotation/1 -> Square/1
  Rotation1/1 -> Product3/2
  Sum of Elements2/1 -> Gain3/1
  Conj/1 -> Product1/2
  Sum of Elements1/1 -> Gain2/1
  Square/1 -> Product2/2
  Sum of Elements3/1 -> Gain4/1
  osc[3]/1 -> Demux/1
  Gain3/1 -> convert_to_LL1/1
  Gain2/1 -> convert_to_LL/1
  in[3]/1 -> Product1/1
  Demux/2 -> Terminator/1
  Demux/3 -> Terminator1/1
  Gain5/1 -> Sum of Elements1/1, Product3/1, Product2/1

== system My_gfm_battery_sil_2/My Inverter Controller /My_acMonitor_A/PLL_3ph ==
  note: cos x - j sin x
      | cos (x-120) - j (sin x -120)
      | cos (x+120) - j (sin x +120)
  note: cos x + j sin x
      | cos (x-120) + j (sin x -120)
      | cos (x+120) + j (sin x +120)
  note: -sin x
      |  -sin (x -120)
      |  -sin (x +120)
  note: Vq
  note: filter 120 Hz, due to negative sequence
  note: Leaky Integrator
  note: vd = Va * cos x + Vb * cos (x-120) + Vc * cos (x+120)
  note: vq = -Va * sin x - Vb * sin (x-120) - Vc * sin (x+120)
  note: Va = vd * cos x - vq * sin x
  note: Vb = vd * cos (x-120) - vq * sin (x-120)
  note: Vc = vd * cos (x+120) - vq * sin (x+120)
  ref : Inport
  Complex to Real-Imag : ComplexToRealImag
  Conj : Math  Operator=conj  SaturateOnIntegerOverflow=on
  Constant : Constant  Value=120
  Gain1 : Gain  Gain=1.5
  Gain2 : Gain  Gain=4.5
  Gain3 : Gain  Gain=10e-3
  Integrator : Integrator  LimitOutput=on  UpperSaturationLimit=5  LowerSaturationLimit=-5
  Product : Product
  SOGI : controls_element_lib/dcVoltageRegulator_A/SOGI  SystemSampleTime=-1
  Saturation : Saturate  UpperLimit=5  LowerLimit=-5
  Sum : Sum  Inputs=+++
  Sum of Elements : Sum  Inputs=+
  Sum1 : Sum  Inputs=|+-
  Terminator : Terminator
  Terminator1 : Terminator
  Transfer Fcn : TransferFcn  Denominator=[0.02 1]
  f_nom : Constant  Value=nominalFrequency
  oscillator_3ph : Subsystem
  osc[3] : Outport  VectorParamsAs1DForOutWhenUnconnected=on
  freq : Outport  Port=2  VectorParamsAs1DForOutWhenUnconnected=on
  wires:
  Constant/1 -> SOGI/2
  Transfer Fcn/1 -> SOGI/1  "phase_error"
  f_nom/1 -> Sum/1
  Gain3/1 -> Sum1/2
  Sum of Elements/1 -> Transfer Fcn/1
  SOGI/1 -> Gain1/1, Gain2/1  "phase_error"
  Saturation/1 -> Sum/2
  Product/1 -> Sum of Elements/1
  Sum/1 -> freq/1, oscillator_3ph/1(f)  "freq"
  oscillator_3ph/1(osc[3]) -> Conj/1, osc[3]/1
  Gain2/1 -> Sum1/1
  Complex to Real-Imag/2 -> Product/2
  Sum1/1 -> Integrator/1
  Integrator/1 -> Gain3/1, Sum/3
  ref/1 -> Product/1
  Conj/1 -> Complex to Real-Imag/1
  Gain1/1 -> Saturation/1
  Complex to Real-Imag/1 -> Terminator/1
  SOGI/2 -> Terminator1/1

== system My_gfm_battery_sil_2/My Inverter Controller /My_acMonitor_A/RMS_Analyzer ==
  in : Inport
  Gain : Gain  Gain=2 * pi * 10
  Integrator : Integrator  InitialCondition=0.01
  Sqrt : Sqrt  SaturateOnIntegerOverflow=on
  Square : Math  Operator=square  SaturateOnIntegerOverflow=on
  Sum : Sum  Inputs=|+-
  RMS : Outport  VectorParamsAs1DForOutWhenUnconnected=on
  wires:
  Square/1 -> Sum/1
  in/1 -> Square/1
  Gain/1 -> Integrator/1
  Sum/1 -> Gain/1
  Integrator/1 -> Sum/2, Sqrt/1
  Sqrt/1 -> RMS/1

== system My_gfm_battery_sil_2/My Inverter Controller /My_acMonitor_A/SOGI ==
  in : Inport
  fnom : Inport  Port=2
  2pi : Gain  Gain=2*pi
  Integrator2 : Integrator
  Integrator3 : Integrator
  Product : Product
  Product1 : Product
  Sum4 : Sum  Inputs=|+-
  Sum5 : Sum  Inputs=|+-
  alpha : Gain  Gain=1 / sqrt(2)
  notch : Outport  VectorParamsAs1DForOutWhenUnconnected=on
  bpf : Outport  Port=2  VectorParamsAs1DForOutWhenUnconnected=on
  wires:
  Product1/1 -> Integrator3/1
  Product/1 -> Integrator2/1
  2pi/1 -> Product/2, Product1/2
  Integrator3/1 -> Sum4/2
  Sum4/1 -> Product/1
  Sum5/1 -> notch/1, alpha/1
  alpha/1 -> Sum4/1
  Integrator2/1 -> bpf/1, Sum5/2, Product1/1
  fnom/1 -> 2pi/1
  in/1 -> Sum5/1

== system My_gfm_battery_sil_2/My Inverter Controller /My_circuit_controls_A/LPF ==
  1 : Inport
  Gain2 : Gain  Gain=1/20e-6
  Integrator : Integrator
  Sum4 : Sum  Inputs=|+-
  Out1 : Outport  VectorParamsAs1DForOutWhenUnconnected=on
  wires:
  Gain2/1 -> Integrator/1
  Integrator/1 -> Sum4/2, Out1/1
  1/1 -> Sum4/1
  Sum4/1 -> Gain2/1

== system My_gfm_battery_sil_2/My Inverter Controller /My_circuit_controls_A/LPF1 ==
  1 : Inport
  Gain2 : Gain  Gain=1/20e-6
  Integrator : Integrator
  Sum4 : Sum  Inputs=|+-
  Out1 : Outport  VectorParamsAs1DForOutWhenUnconnected=on
  wires:
  Gain2/1 -> Integrator/1
  Integrator/1 -> Sum4/2, Out1/1
  1/1 -> Sum4/1
  Sum4/1 -> Gain2/1

== system My_gfm_battery_sil_2/My Inverter Controller /My_circuit_controls_A/LPF2 ==
  1 : Inport
  Gain2 : Gain  Gain=1/20e-6
  Integrator : Integrator
  Sum4 : Sum  Inputs=|+-
  Out1 : Outport  VectorParamsAs1DForOutWhenUnconnected=on
  wires:
  Sum4/1 -> Gain2/1
  1/1 -> Sum4/1
  Integrator/1 -> Out1/1, Sum4/2
  Gain2/1 -> Integrator/1

== system My_gfm_battery_sil_2/My Inverter Controller /My_circuit_controls_A/LPF3 ==
  1 : Inport
  Gain2 : Gain  Gain=1/500e-6
  Integrator : Integrator
  Sum4 : Sum  Inputs=|+-
  Out1 : Outport  VectorParamsAs1DForOutWhenUnconnected=on
  wires:
  Gain2/1 -> Integrator/1
  Integrator/1 -> Sum4/2, Out1/1
  1/1 -> Sum4/1
  Sum4/1 -> Gain2/1

== system My_gfm_battery_sil_2/My Inverter Controller /My_circuit_controls_A/SOGI_BPF ==
  in : Inport
  f : Inport  Port=2
  Gain : Gain
  Gain2 : Gain  Gain=2*pi
  Integrator : Integrator
  Integrator1 : Integrator
  Product : Product
  Product2 : Product
  Sum : Sum  Inputs=|+-
  Sum1 : Sum  Inputs=|+-
  Notched : Outport  VectorParamsAs1DForOutWhenUnconnected=on
  wires:
  f/1 -> Gain2/1
  in/1 -> Sum1/1
  Product/1 -> Integrator/1
  Integrator1/1 -> Product2/1
  Gain/1 -> Sum1/2
  Sum1/1 -> Notched/1, Sum/1
  Integrator/1 -> Integrator1/1, Gain/1
  Gain2/1 -> Product2/2, Product/2
  Sum/1 -> Product/1
  Product2/1 -> Sum/2

== system My_gfm_battery_sil_2/My Inverter Controller /My_circuit_controls_A/virtual damper ==
  v : Inport
  1/tau_damp : Gain  Gain=1/250e-6
  Integrator : Integrator
  Sum : Sum  Inputs=|+-
  g_damp : Gain  Gain=1/(0.8*Z_INV_BASE)
  i_damp : Outport  VectorParamsAs1DForOutWhenUnconnected=on
  wires:
  g_damp/1 -> i_damp/1
  Sum/1 -> g_damp/1, 1/tau_damp/1
  v/1 -> Sum/1
  1/tau_damp/1 -> Integrator/1
  Integrator/1 -> Sum/2

== system My_gfm_battery_sil_2/My Inverter Controller /My_circuit_controls_A1/LPF ==
  1 : Inport
  Gain2 : Gain  Gain=1/20e-6
  Integrator : Integrator
  Sum4 : Sum  Inputs=|+-
  Out1 : Outport  VectorParamsAs1DForOutWhenUnconnected=on
  wires:
  Gain2/1 -> Integrator/1
  Integrator/1 -> Sum4/2, Out1/1
  1/1 -> Sum4/1
  Sum4/1 -> Gain2/1

== system My_gfm_battery_sil_2/My Inverter Controller /My_circuit_controls_A1/LPF1 ==
  1 : Inport
  Gain2 : Gain  Gain=1/20e-6
  Integrator : Integrator
  Sum4 : Sum  Inputs=|+-
  Out1 : Outport  VectorParamsAs1DForOutWhenUnconnected=on
  wires:
  Gain2/1 -> Integrator/1
  Integrator/1 -> Sum4/2, Out1/1
  1/1 -> Sum4/1
  Sum4/1 -> Gain2/1

== system My_gfm_battery_sil_2/My Inverter Controller /My_circuit_controls_A1/LPF2 ==
  1 : Inport
  Gain2 : Gain  Gain=1/20e-6
  Integrator : Integrator
  Sum4 : Sum  Inputs=|+-
  Out1 : Outport  VectorParamsAs1DForOutWhenUnconnected=on
  wires:
  Sum4/1 -> Gain2/1
  1/1 -> Sum4/1
  Integrator/1 -> Out1/1, Sum4/2
  Gain2/1 -> Integrator/1

== system My_gfm_battery_sil_2/My Inverter Controller /My_circuit_controls_A1/SOGI_BPF ==
  in : Inport
  f : Inport  Port=2
  Gain : Gain
  Gain2 : Gain  Gain=2*pi
  Integrator : Integrator
  Integrator1 : Integrator
  Product : Product
  Product2 : Product
  Sum : Sum  Inputs=|+-
  Sum1 : Sum  Inputs=|+-
  Notched : Outport  VectorParamsAs1DForOutWhenUnconnected=on
  wires:
  f/1 -> Gain2/1
  in/1 -> Sum1/1
  Product/1 -> Integrator/1
  Integrator1/1 -> Product2/1
  Gain/1 -> Sum1/2
  Sum1/1 -> Notched/1, Sum/1
  Integrator/1 -> Integrator1/1, Gain/1
  Gain2/1 -> Product2/2, Product/2
  Sum/1 -> Product/1
  Product2/1 -> Sum/2

== system My_gfm_battery_sil_2/My Inverter Controller /My_circuit_controls_A1/virtual damper ==
  v : Inport
  1/tau_damp : Gain  Gain=1/250e-6
  Integrator : Integrator
  Sum : Sum  Inputs=|+-
  g_damp : Gain  Gain=1/(0.8*Z_INV_BASE)
  i_damp : Outport  VectorParamsAs1DForOutWhenUnconnected=on
  wires:
  g_damp/1 -> i_damp/1
  Sum/1 -> g_damp/1, 1/tau_damp/1
  v/1 -> Sum/1
  1/tau_damp/1 -> Integrator/1
  Integrator/1 -> Sum/2

== system My_gfm_battery_sil_2/My Inverter Controller /My_currentLimiting_B/Current_foldback1 ==
  V[3]_pu : Inport
  Vmax : Inport  Port=2
  Abs1 : Abs
  Constant1 : Constant
  Gain : Gain  Gain=5
  "LPF " : Subsystem
  Max : MinMax  Function=max
  Saturation : Saturate  UpperLimit=1  LowerLimit=0.05
  Scope1 : Scope  NumInputPorts=3
  Sum1 : Sum  Inputs=|+-
  Sum2 : Sum  Inputs=|++
  Transfer Fcn : TransferFcn  Denominator=[0.01 1]
  limit_pu : Outport  VectorParamsAs1DForOutWhenUnconnected=on
  wires:
  "LPF "/1(Out) -> Gain/1
  V[3]_pu/1 -> Abs1/1
  Sum2/1 -> Saturation/1
  Constant1/1 -> Sum2/2
  Vmax/1 -> Scope1/1, Sum1/1
  Saturation/1 -> limit_pu/1
  Abs1/1 -> Max/1
  Max/1 -> Sum1/2, Scope1/3
  Sum1/1 -> "LPF "/1(In), Scope1/2
  Gain/1 -> Sum2/1

== system My_gfm_battery_sil_2/My Inverter Controller /My_currentLimiting_B/RMS_Analyzer ==
  in : Inport
  Gain : Gain  Gain=1/0.02
  Integrator : Integrator
  Sqrt : Sqrt  SaturateOnIntegerOverflow=on
  Square : Math  Operator=square  SaturateOnIntegerOverflow=on
  Sum : Sum  Inputs=|+-
  RMS : Outport  VectorParamsAs1DForOutWhenUnconnected=on
  wires:
  Square/1 -> Sum/1
  in/1 -> Square/1
  Gain/1 -> Integrator/1
  Sum/1 -> Gain/1
  Integrator/1 -> Sum/2, Sqrt/1
  Sqrt/1 -> RMS/1

== system My_gfm_battery_sil_2/My Inverter Controller /My_currentLimiting_B/RMS_Analyzer1 ==
  in : Inport
  Gain : Gain  Gain=1/0.02
  Integrator : Integrator
  Sqrt : Sqrt  SaturateOnIntegerOverflow=on
  Square : Math  Operator=square  SaturateOnIntegerOverflow=on
  Sum : Sum  Inputs=|+-
  RMS : Outport  VectorParamsAs1DForOutWhenUnconnected=on
  wires:
  Square/1 -> Sum/1
  in/1 -> Square/1
  Gain/1 -> Integrator/1
  Sum/1 -> Gain/1
  Integrator/1 -> Sum/2, Sqrt/1
  Sqrt/1 -> RMS/1

== system My_gfm_battery_sil_2/My Inverter Controller /My_currentLimiting_B/SOGI_BPF ==
  in : Inport
  f : Inport  Port=2
  Gain : Gain
  Gain2 : Gain  Gain=2*pi
  Integrator : Integrator
  Integrator1 : Integrator
  Product : Product
  Product2 : Product
  Sum : Sum  Inputs=|+-
  Sum1 : Sum  Inputs=|+-
  bpf : Outport  VectorParamsAs1DForOutWhenUnconnected=on
  wires:
  f/1 -> Gain2/1
  in/1 -> Sum1/1
  Product/1 -> Integrator/1
  Integrator1/1 -> Product2/1
  Gain/1 -> Sum1/2
  Sum1/1 -> Sum/1
  Integrator/1 -> Integrator1/1, Gain/1, bpf/1
  Gain2/1 -> Product2/2, Product/2
  Sum/1 -> Product/1
  Product2/1 -> Sum/2

== system My_gfm_battery_sil_2/My Inverter Controller /My_currentLimiting_B/estimate_excess ==
  note: why?
  note: Iabc rms
  Ilimit : Inport
  I[3] : Inport  Port=2
  Abs1 : Abs
  Constant : Constant
  Max : MinMax  Function=max
  Min : MinMax  Function=max  Inputs=2
  Product1 : Product  Inputs=*/
  Scope11 : Scope  NumInputPorts=4
  Sum : Sum  Inputs=|+-
  excess_fraction : Outport  VectorParamsAs1DForOutWhenUnconnected=on
  wires:
  Sum/1 -> excess_fraction/1
  Constant/1 -> Sum/1
  Product1/1 -> Sum/2  "scale_factor"
  Max/1 -> Scope11/3, Min/2  "max_Iph"
  Ilimit/1 -> Scope11/1, Product1/1, Min/1  "Irms_limit"
  Abs1/1 -> Max/1
  I[3]/1 -> Scope11/4, Abs1/1
  Min/1 -> Scope11/2, Product1/2

== system My_gfm_battery_sil_2/My Inverter Controller /My_currentLimiting_B/soft_saturation ==
  note: 1-e(-dx/H)
  note: dX
  note: dX/Xau
  note: -1+e(-dx/H)
  note: H*[1-e(-dx/H)] + H*[-1+e(-dx/H)]
  in : Inport
  Constant : Constant
  Constant1 : Constant
  Exp : Math  SaturateOnIntegerOverflow=on
  Exp1 : Math  SaturateOnIntegerOverflow=on
  Gain : Gain  Gain=-1
  Gain1 : Gain  Gain=Xau
  Product : Product  Inputs=*/
  Sum : Sum  Inputs=|++
  Sum1 : Sum  Inputs=-+|
  Sum2 : Sum  Inputs=|+-
  Sum3 : Sum  Inputs=|+-
  Sum4 : Sum  Inputs=|++
  headroom : Gain  Gain=(hard_limit - soft_limit)
  headroom1 : Constant  Value=max(hard_limit - soft_limit, 1e-3)
  negative : Saturate  UpperLimit=0  LowerLimit=-inf
  positive : Saturate  UpperLimit=inf  LowerLimit=0
  soft_limit : Saturate  UpperLimit=soft_limit  LowerLimit=-soft_limit
  out : Outport  VectorParamsAs1DForOutWhenUnconnected=on
  wires:
  headroom1/1 -> Gain1/1
  Sum1/1 -> Product/1
  Sum2/1 -> Sum4/1
  Sum4/1 -> headroom/1
  Gain/1 -> Exp/1
  headroom/1 -> Sum/2
  Exp/1 -> Sum2/2
  positive/1 -> Gain/1
  in/1 -> soft_limit/1, Sum1/2
  Exp1/1 -> Sum3/1
  Sum/1 -> out/1
  soft_limit/1 -> Sum1/1, Sum/1
  Sum3/1 -> Sum4/2
  negative/1 -> Exp1/1
  Constant1/1 -> Sum3/2
  Product/1 -> positive/1, negative/1
  Constant/1 -> Sum2/1
  Gain1/1 -> Product/2  "Xau"

== system My_gfm_battery_sil_2/My Inverter Controller /My_currentLimiting_B/soft_saturation1 ==
  in : Inport
  Constant : Constant
  Constant1 : Constant
  Exp : Math  SaturateOnIntegerOverflow=on
  Exp1 : Math  SaturateOnIntegerOverflow=on
  Gain : Gain  Gain=-1
  Product : Product  Inputs=*/
  Sum : Sum  Inputs=|++
  Sum1 : Sum  Inputs=-+|
  Sum2 : Sum  Inputs=|+-
  Sum3 : Sum  Inputs=|+-
  Sum4 : Sum  Inputs=|++
  headroom : Gain  Gain=(hard_limit - soft_limit)
  headroom1 : Constant  Value=max(hard_limit - soft_limit, 1e-3)
  negative : Saturate  UpperLimit=0  LowerLimit=-inf
  positive : Saturate  UpperLimit=inf  LowerLimit=0
  soft_limit : Saturate  UpperLimit=soft_limit  LowerLimit=-soft_limit
  out : Outport  VectorParamsAs1DForOutWhenUnconnected=on
  wires:
  headroom1/1 -> Product/2
  Sum1/1 -> Product/1
  Sum2/1 -> Sum4/1
  Sum4/1 -> headroom/1
  Gain/1 -> Exp/1
  headroom/1 -> Sum/2
  Exp/1 -> Sum2/2
  positive/1 -> Gain/1
  in/1 -> soft_limit/1, Sum1/2
  Exp1/1 -> Sum3/1
  Sum/1 -> out/1
  soft_limit/1 -> Sum1/1, Sum/1
  Sum3/1 -> Sum4/2
  negative/1 -> Exp1/1
  Constant1/1 -> Sum3/2
  Product/1 -> positive/1, negative/1
  Constant/1 -> Sum2/1

== system My_gfm_battery_sil_2/My Inverter Controller /My_currentLimiting_B1/RMS_Analyzer ==
  in : Inport
  Gain : Gain  Gain=1/0.02
  Integrator : Integrator
  Sqrt : Sqrt  SaturateOnIntegerOverflow=on
  Square : Math  Operator=square  SaturateOnIntegerOverflow=on
  Sum : Sum  Inputs=|+-
  RMS : Outport  VectorParamsAs1DForOutWhenUnconnected=on
  wires:
  Square/1 -> Sum/1
  in/1 -> Square/1
  Gain/1 -> Integrator/1
  Sum/1 -> Gain/1
  Integrator/1 -> Sum/2, Sqrt/1
  Sqrt/1 -> RMS/1

== system My_gfm_battery_sil_2/My Inverter Controller /My_currentLimiting_B1/SOGI_BPF ==
  in : Inport
  f : Inport  Port=2
  Gain : Gain
  Gain2 : Gain  Gain=2*pi
  Integrator : Integrator
  Integrator1 : Integrator
  Product : Product
  Product2 : Product
  Sum : Sum  Inputs=|+-
  Sum1 : Sum  Inputs=|+-
  bpf : Outport  VectorParamsAs1DForOutWhenUnconnected=on
  wires:
  f/1 -> Gain2/1
  in/1 -> Sum1/1
  Product/1 -> Integrator/1
  Integrator1/1 -> Product2/1
  Gain/1 -> Sum1/2
  Sum1/1 -> Sum/1
  Integrator/1 -> Integrator1/1, Gain/1, bpf/1
  Gain2/1 -> Product2/2, Product/2
  Sum/1 -> Product/1
  Product2/1 -> Sum/2

== system My_gfm_battery_sil_2/My Inverter Controller /My_currentLimiting_B1/estimate_excess ==
  note: why?
  note: Iabc rms
  Ilimit : Inport
  I[3] : Inport  Port=2
  Abs1 : Abs
  Constant : Constant
  Max : MinMax  Function=max
  Min : MinMax  Function=max  Inputs=2
  Product1 : Product  Inputs=*/
  Scope11 : Scope  NumInputPorts=4
  Sum : Sum  Inputs=|+-
  excess_fraction : Outport  VectorParamsAs1DForOutWhenUnconnected=on
  wires:
  Sum/1 -> excess_fraction/1
  Constant/1 -> Sum/1
  Product1/1 -> Sum/2  "scale_factor"
  Max/1 -> Scope11/3, Min/2  "max_Iph"
  Ilimit/1 -> Scope11/1, Product1/1, Min/1  "Irms_limit"
  Abs1/1 -> Max/1
  I[3]/1 -> Scope11/4, Abs1/1
  Min/1 -> Scope11/2, Product1/2

== system My_gfm_battery_sil_2/My Inverter Controller /My_currentLimiting_B1/soft_saturation ==
  note: 1-e(-dx/H)
  note: dX
  note: dX/Xau
  note: -1+e(-dx/H)
  note: H*[1-e(-dx/H)] + H*[-1+e(-dx/H)]
  in : Inport
  Constant : Constant
  Constant1 : Constant
  Exp : Math  SaturateOnIntegerOverflow=on
  Exp1 : Math  SaturateOnIntegerOverflow=on
  Gain : Gain  Gain=-1
  Gain1 : Gain  Gain=Xau
  Product : Product  Inputs=*/
  Sum : Sum  Inputs=|++
  Sum1 : Sum  Inputs=-+|
  Sum2 : Sum  Inputs=|+-
  Sum3 : Sum  Inputs=|+-
  Sum4 : Sum  Inputs=|++
  headroom : Gain  Gain=(hard_limit - soft_limit)
  headroom1 : Constant  Value=max(hard_limit - soft_limit, 1e-3)
  negative : Saturate  UpperLimit=0  LowerLimit=-inf
  positive : Saturate  UpperLimit=inf  LowerLimit=0
  soft_limit : Saturate  UpperLimit=soft_limit  LowerLimit=-soft_limit
  out : Outport  VectorParamsAs1DForOutWhenUnconnected=on
  wires:
  headroom1/1 -> Gain1/1
  Sum1/1 -> Product/1
  Sum2/1 -> Sum4/1
  Sum4/1 -> headroom/1
  Gain/1 -> Exp/1
  headroom/1 -> Sum/2
  Exp/1 -> Sum2/2
  positive/1 -> Gain/1
  in/1 -> soft_limit/1, Sum1/2
  Exp1/1 -> Sum3/1
  Sum/1 -> out/1
  soft_limit/1 -> Sum1/1, Sum/1
  Sum3/1 -> Sum4/2
  negative/1 -> Exp1/1
  Constant1/1 -> Sum3/2
  Product/1 -> positive/1, negative/1
  Constant/1 -> Sum2/1
  Gain1/1 -> Product/2  "Xau"

== system My_gfm_battery_sil_2/My Inverter Controller /My_currentLimiting_B1/soft_saturation1 ==
  in : Inport
  Constant : Constant
  Constant1 : Constant
  Exp : Math  SaturateOnIntegerOverflow=on
  Exp1 : Math  SaturateOnIntegerOverflow=on
  Gain : Gain  Gain=-1
  Product : Product  Inputs=*/
  Sum : Sum  Inputs=|++
  Sum1 : Sum  Inputs=-+|
  Sum2 : Sum  Inputs=|+-
  Sum3 : Sum  Inputs=|+-
  Sum4 : Sum  Inputs=|++
  headroom : Gain  Gain=(hard_limit - soft_limit)
  headroom1 : Constant  Value=max(hard_limit - soft_limit, 1e-3)
  negative : Saturate  UpperLimit=0  LowerLimit=-inf
  positive : Saturate  UpperLimit=inf  LowerLimit=0
  soft_limit : Saturate  UpperLimit=soft_limit  LowerLimit=-soft_limit
  out : Outport  VectorParamsAs1DForOutWhenUnconnected=on
  wires:
  headroom1/1 -> Product/2
  Sum1/1 -> Product/1
  Sum2/1 -> Sum4/1
  Sum4/1 -> headroom/1
  Gain/1 -> Exp/1
  headroom/1 -> Sum/2
  Exp/1 -> Sum2/2
  positive/1 -> Gain/1
  in/1 -> soft_limit/1, Sum1/2
  Exp1/1 -> Sum3/1
  Sum/1 -> out/1
  soft_limit/1 -> Sum1/1, Sum/1
  Sum3/1 -> Sum4/2
  negative/1 -> Exp1/1
  Constant1/1 -> Sum3/2
  Product/1 -> positive/1, negative/1
  Constant/1 -> Sum2/1

== system My_gfm_battery_sil_2/My Inverter Controller /My_currentSource_A/current_modulator ==
  I_cmd : Inport
  osc : Inport  Port=2
  Complex to Real-Imag : ComplexToRealImag
  Complex to Real-Imag1 : ComplexToRealImag
  Gain : Gain  Gain=sqrt(2)
  Product1 : Product
  Product2 : Product
  Sum1 : Sum  Inputs=|+-
  i_ref : Outport  VectorParamsAs1DForOutWhenUnconnected=on
  wires:
  osc/1 -> Gain/1
  Complex to Real-Imag/1 -> Product2/2
  Product2/1 -> Sum1/1
  Sum1/1 -> i_ref/1  "i"
  Gain/1 -> Complex to Real-Imag/1
  Complex to Real-Imag/2 -> Product1/2
  Product1/1 -> Sum1/2
  I_cmd/1 -> Complex to Real-Imag1/1
  Complex to Real-Imag1/1 -> Product2/1
  Complex to Real-Imag1/2 -> Product1/1
